simulink model "Highway_Assist"  (R2021a)
settings: Solver=VariableStepAuto  StartTime=0.0  StopTime=100  RelTol=1e-3
values from neighbouring files (symbols this model uses):
  Cf = 155494.663    [Highway_Assist_init.m]
  Cr = 1554494.663    [Highway_Assist_init.m]
  Iz = 1436.24    [Highway_Assist_init.m]
  lf = 1.165    [Highway_Assist_init.m]
  lr = 1.165    [Highway_Assist_init.m]
  m = 1140    [Highway_Assist_init.m]
  md = get_curvature(Vx, yaw_rate_pose, tRef)    [Highway_Assist_init.m]
  Ts = 0.1    [Highway_Assist_init.m]
  V_init = Vx    (= 25)    [Highway_Assist_init.m]
undefined symbols (not defined in the file or in its folder): sigbuilder_block
libraries: pid_lib x2, mpcadaslib x1
(part 1 of 2)
settings Model: Creator=User  LastModifiedBy=User

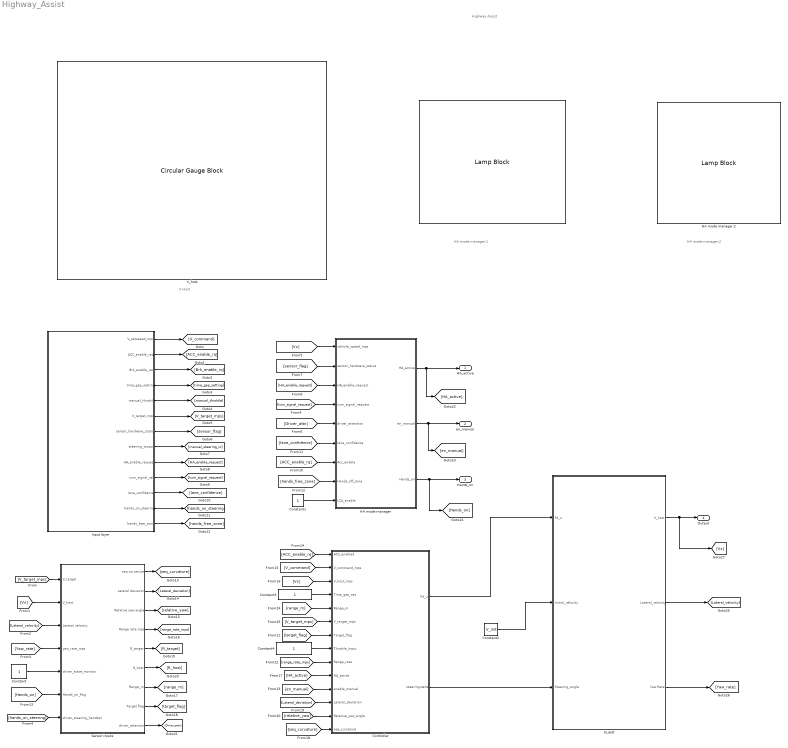
== system Highway_Assist ==
  note: HA mode manager:2
  note: V Host
  note: HA mode manager:1
  note: Highway Assist
  " " : LampBlock
  Constant{,1,3..4} (4 alike) : Constant
  Constant2 : Constant  Value=V_init
  Controller : Subsystem
  HA mode manager : Subsystem
  HA mode manager:2 : LampBlock
  Input layer : Subsystem
  PLANT : Subsystem
  Sensor inputs : Subsystem
  V_host : CircularGaugeBlock
  HA_active : Outport
  en_manual : Outport  Port=2
  Hands_on : Outport  Port=3
  Output : Outport  Port=4
  wires:
  Input layer/1(V_setspeed_mps) -> [V_command]
  Input layer/2(ACC_enable_req) -> [ACC_enable_rq]
  Input layer/3(Brk_enable_req) -> [Brk_enable_rq]
  Input layer/4(time_gap_setting) -> [time_gap_setting]
  Input layer/5(manual_throttle) -> [manual_throttle]
  Input layer/6(V_target_mps) -> [V_target_mps]
  Input layer/7(sensor_hardware_status) -> [sensor_flag]
  Input layer/8(steering_torque) -> [manual_steering_io]
  Input layer/9(HA_enable_request) -> [HA_enable_request]
  Input layer/10(turn_signal_req) -> [turn_signal_request]
  Input layer/11(lane_confidence) -> [lane_confidence]
  Input layer/12(hands_on_steering) -> [hands_on_steering]
  Input layer/13(hands_free_zone) -> [hands_free_zone]
  [V_target_mps] -> Sensor inputs/1(V_target)
  [Vx] -> Sensor inputs/2(V_host)
  [Lateral_velocity] -> Sensor inputs/3(Lateral velocity)
  [Yaw_rate] -> Sensor inputs/4(yaw_rate_mps)
  Constant/1 -> Sensor inputs/5(driver_state_monitor)
  [hands_on_steering] -> Sensor inputs/7(driver_steering_handson)
  [Vx] -> HA mode manager/1(vehicle_speed_mps)
  Sensor inputs/1(seq curvature) -> [seq_curvature]
  Sensor inputs/2(Lateral deviation) -> [Lateral_deviation]
  Sensor inputs/3(Relative yaw angle) -> [relative_yaw]
  Sensor inputs/4(Range rate mps) -> [range_rate_mps]
  Sensor inputs/7(Range_m) -> [range_m]
  Sensor inputs/8(Target flag) -> [target_flag]
  Sensor inputs/5(R_target) -> [R_target]
  Sensor inputs/6(R_host) -> [R_host]
  Sensor inputs/9(driver_attention) -> [Driver_attn]
  [Driver_attn] -> HA mode manager/5(driver_attention)
  [sensor_flag] -> HA mode manager/2(sensor_hardware_status)
  [HA_enable_request] -> HA mode manager/3(HA_enable_request)
  [turn_signal_request] -> HA mode manager/4(turn_signal_request)
  Constant1/1 -> HA mode manager/9(LCA_enable)
  [ACC_enable_rq] -> HA mode manager/7(Acc_enable)
  [lane_confidence] -> HA mode manager/6(lane_confidence)
  [hands_free_zone] -> HA mode manager/8(Hands_off_zone)
  HA mode manager/1(HA_active) -> [HA_active], HA_active/1
  HA mode manager/2(en_manual) -> [en_manual], en_manual/1
  HA mode manager/3(Hands_on) -> [Hands_on], Hands_on/1
  [Hands_on] -> Sensor inputs/6(Hands_on_flag)
  [ACC_enable_rq] -> Controller/1(ACC_enabled)
  [V_command] -> Controller/2(V_command_mps)
  [Vx] -> Controller/3(V_host_mps)
  Controller/1(Fd_u) -> PLANT/1(Fd_u)
  Controller/2(steering-delta) -> PLANT/3(Steering_angle)
  Constant2/1 -> PLANT/2(Initial_velocity)
  [HA_active] -> Controller/10(HA_active)
  [seq_curvature] -> Controller/14(seq_curvature)
  [Lateral_deviation] -> Controller/12(Lateral_deviation)
  [relative_yaw] -> Controller/13(Relative_yaw_angle)
  [target_flag] -> Controller/7(Target_flag)
  [range_rate_mps] -> Controller/9(Range_rate)
  [en_manual] -> Controller/11(enable_manual)
  [range_m] -> Controller/5(Range_m)
  [V_target_mps] -> Controller/6(V_target_mps)
  PLANT/2(Lateral_velocity) -> [Lateral_velocity]
  PLANT/3(Yaw Rate) -> [Yaw_rate]
  PLANT/1(V_host) -> Output/1, [Vx]
  Constant3/1 -> Controller/4(Time_gap_sec)
  Constant4/1 -> Controller/8(Throttle_input)

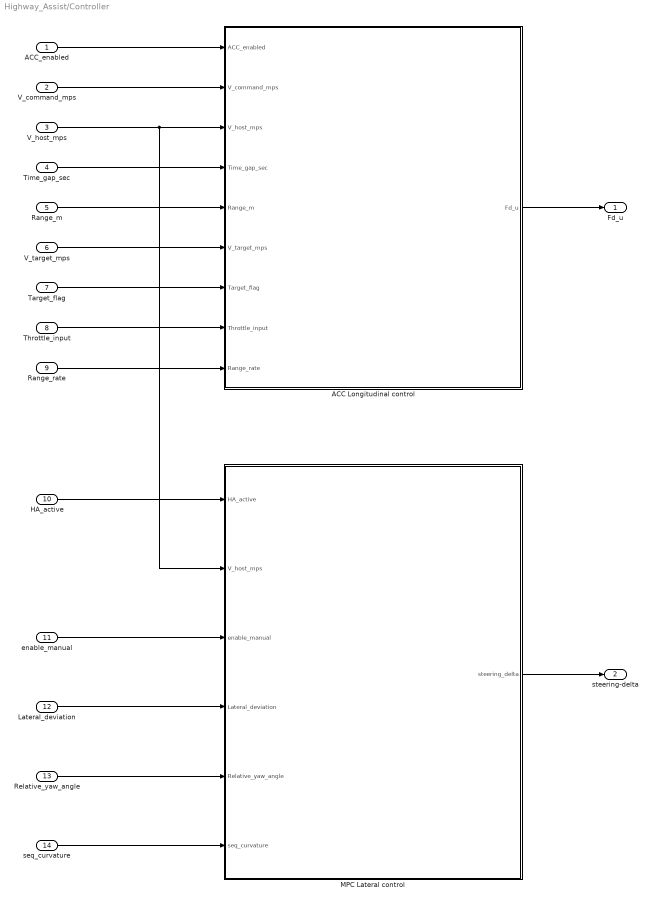
== system Highway_Assist/Controller ==
  ACC_enabled : Inport
  V_command_mps : Inport  Port=2
  V_host_mps : Inport  Port=3
  Time_gap_sec : Inport  Port=4
  Range_m : Inport  Port=5
  V_target_mps : Inport  Port=6
  Target_flag : Inport  Port=7
  Throttle_input : Inport  Port=8
  Range_rate : Inport  Port=9
  HA_active : Inport  Port=10
  enable_manual : Inport  Port=11
  Lateral_deviation : Inport  Port=12
  Relative_yaw_angle : Inport  Port=13
  seq_curvature : Inport  Port=14
  ACC Longitudinal control : Subsystem
  MPC Lateral control : Subsystem
  Fd_u : Outport
  steering-delta : Outport  Port=2
  wires:
  ACC_enabled/1 -> ACC Longitudinal control/1(ACC_enabled)
  V_command_mps/1 -> ACC Longitudinal control/2(V_command_mps)
  Time_gap_sec/1 -> ACC Longitudinal control/4(Time_gap_sec)
  Range_m/1 -> ACC Longitudinal control/5(Range_m)
  V_target_mps/1 -> ACC Longitudinal control/6(V_target_mps)
  Target_flag/1 -> ACC Longitudinal control/7(Target_flag)
  Throttle_input/1 -> ACC Longitudinal control/8(Throttle_input)
  Range_rate/1 -> ACC Longitudinal control/9(Range_rate)
  ACC Longitudinal control/1(Fd_u) -> Fd_u/1
  MPC Lateral control/1(steering_delta) -> steering-delta/1
  V_host_mps/1 -> MPC Lateral control/2(V_host_mps), ACC Longitudinal control/3(V_host_mps)
  HA_active/1 -> MPC Lateral control/1(HA_active)
  enable_manual/1 -> MPC Lateral control/3(enable_manual)
  Lateral_deviation/1 -> MPC Lateral control/4(Lateral_deviation)
  Relative_yaw_angle/1 -> MPC Lateral control/5(Relative_yaw_angle)
  seq_curvature/1 -> MPC Lateral control/6(seq_curvature)

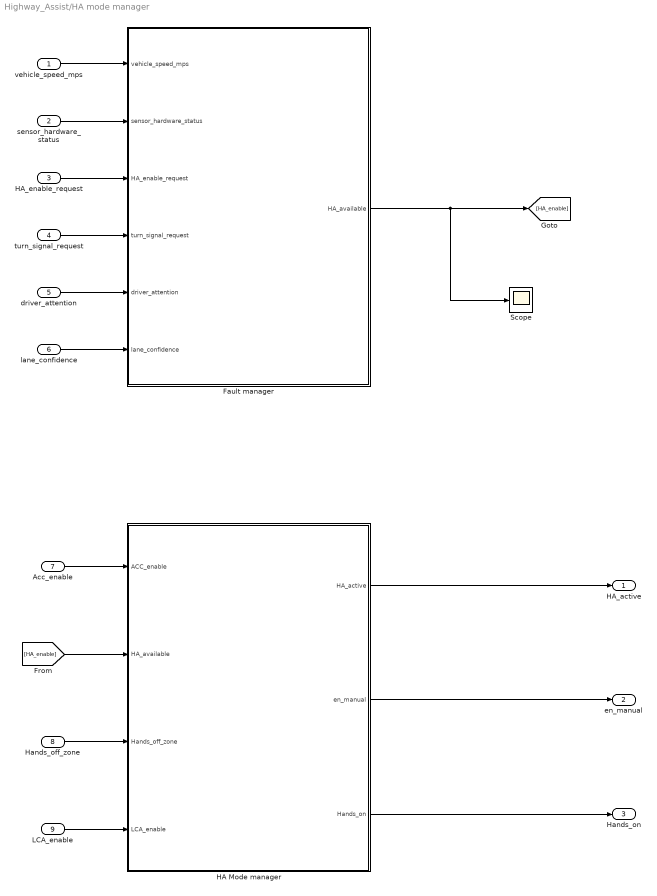
== system Highway_Assist/HA mode manager ==
  vehicle_speed_mps : Inport
  sensor_hardware_status : Inport  Port=2
  HA_enable_request : Inport  Port=3
  turn_signal_request : Inport  Port=4
  driver_attention : Inport  Port=5
  lane_confidence : Inport  Port=6
  Acc_enable : Inport  Port=7
  Hands_off_zone : Inport  Port=8
  LCA_enable : Inport  Port=9
  Fault manager : Subsystem
  HA Mode manager : Subsystem
  Scope : Scope
  HA_active : Outport
  en_manual : Outport  Port=2
  Hands_on : Outport  Port=3
  wires:
  vehicle_speed_mps/1 -> Fault manager/1(vehicle_speed_mps)
  sensor_hardware_status/1 -> Fault manager/2(sensor_hardware_status)
  HA_enable_request/1 -> Fault manager/3("\tHA_enable_request")
  turn_signal_request/1 -> Fault manager/4("\tturn_signal_request")
  driver_attention/1 -> Fault manager/5("\tdriver_attention")
  lane_confidence/1 -> Fault manager/6("\tlane_confidence")
  Acc_enable/1 -> HA Mode manager/1(ACC_enable)
  [HA_enable] -> HA Mode manager/2(HA_available)
  Hands_off_zone/1 -> HA Mode manager/3(Hands_off_zone)
  LCA_enable/1 -> HA Mode manager/4(LCA_enable)
  HA Mode manager/1(HA_active) -> HA_active/1
  HA Mode manager/2(en_manual) -> en_manual/1
  HA Mode manager/3(Hands_on) -> Hands_on/1
  Fault manager/1(HA_available) -> Scope/1, [HA_enable]

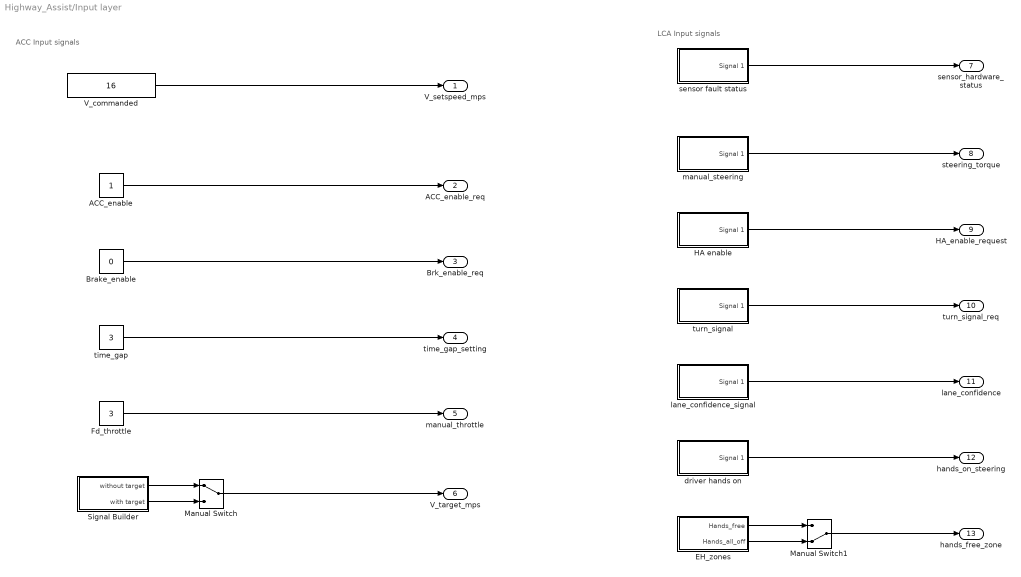
== system Highway_Assist/Input layer ==
  note: LCA Input signals
  note: ACC Input signals
  ACC_enable : Constant
  Brake_enable : Constant  Value=0
  EH_zones : Subsystem  Tag=STV Subsys  LoadFcn=sigbuilder_block('load');  StartFcn=sigbuilder_block('start');  StopFcn=sigbuilder_block('stop');  ClipboardFcn=sigbuilder_block('clipboard');  mask(Sigbuilder block){tuvar=[0:10]}
      mask help: Simulink:masks:SigbuilderBlock_MD
      mask init:
      | if ~strcmp(get_param(bdroot(gcbh),'SimulationStatus'),'stopped') tuvar = sigbuilder_block('maskInit'); end
      settings: CopyFcn=sigbuilder_block('copy');  DeleteFcn=sigbuilder_block('delete');  ModelCloseFcn=sigbuilder_block('modelClose');  PreSaveFcn=sigbuilder_block('preSave');  PauseFcn=sigbuilder_block('pause');  ContinueFcn=sigbuilder_block('continue');  NameChangeFcn=sigbuilder_block('namechange');  OpenFcn=sigbuilder_block('open',[320.25 248.25 550.5 359.25 ]);  CloseFcn=sigbuilder_block('close');
      mask Display: plot(0, 0, 100, 100,[2, 2, 32, 32, 2], [68, 8, 8, 68, 68],[32, 2], [38, 38], [32, 19, 2],[53, 60, 44], [32, 17, 17, 2],[16, 16, 31, 31]);txt = getActiveGroup(gcbh);text(2, 100, txt,'verticalAlignment', 'top');
  Fd_throttle : Constant  Value=3
  HA enable : Subsystem  Tag=STV Subsys  LoadFcn=sigbuilder_block('load');  StartFcn=sigbuilder_block('start');  StopFcn=sigbuilder_block('stop');  ClipboardFcn=sigbuilder_block('clipboard');  mask(Sigbuilder block){tuvar=[0:10]}
      mask help: Simulink:masks:SigbuilderBlock_MD
      mask init:
      | if ~strcmp(get_param(bdroot(gcbh),'SimulationStatus'),'stopped') tuvar = sigbuilder_block('maskInit'); end
      settings: CopyFcn=sigbuilder_block('copy');  DeleteFcn=sigbuilder_block('delete');  ModelCloseFcn=sigbuilder_block('modelClose');  PreSaveFcn=sigbuilder_block('preSave');  PauseFcn=sigbuilder_block('pause');  ContinueFcn=sigbuilder_block('continue');  NameChangeFcn=sigbuilder_block('namechange');  OpenFcn=sigbuilder_block('open',[437.6 199.2 550.4 400 ]);  CloseFcn=sigbuilder_block('close');
      mask Display: plot(0, 0, 100, 100,[2, 2, 32, 32, 2], [68, 8, 8, 68, 68],[32, 2], [38, 38], [32, 19, 2],[53, 60, 44], [32, 17, 17, 2],[16, 16, 31, 31]);txt = getActiveGroup(gcbh);text(2, 100, txt,'verticalAlignment', 'top');
  Manual Switch : ManualSwitch
  Manual Switch1 : ManualSwitch  CurrentSetting=0
  Signal Builder : Subsystem  Tag=STV Subsys  LoadFcn=sigbuilder_block('load');  StartFcn=sigbuilder_block('start');  StopFcn=sigbuilder_block('stop');  ClipboardFcn=sigbuilder_block('clipboard');  mask(Sigbuilder block){tuvar=[0:10]}
      mask help: Simulink:masks:SigbuilderBlock_MD
      mask init:
      | if ~strcmp(get_param(bdroot(gcbh),'SimulationStatus'),'stopped') tuvar = sigbuilder_block('maskInit'); end
      settings: CopyFcn=sigbuilder_block('copy');  DeleteFcn=sigbuilder_block('delete');  ModelCloseFcn=sigbuilder_block('modelClose');  PreSaveFcn=sigbuilder_block('preSave');  PauseFcn=sigbuilder_block('pause');  ContinueFcn=sigbuilder_block('continue');  NameChangeFcn=sigbuilder_block('namechange');  OpenFcn=sigbuilder_block('open',[299.25 217.5 550.5 359.25 ]);  CloseFcn=sigbuilder_block('close');
      mask Display: plot(0, 0, 100, 100,[2, 2, 32, 32, 2], [68, 8, 8, 68, 68],[32, 2], [38, 38], [32, 19, 2],[53, 60, 44], [32, 17, 17, 2],[16, 16, 31, 31]);txt = getActiveGroup(gcbh);text(2, 100, txt,'verticalAlignment', 'top');
  V_commanded : Constant  Value=16
  driver hands on : Subsystem  Tag=STV Subsys  LoadFcn=sigbuilder_block('load');  StartFcn=sigbuilder_block('start');  StopFcn=sigbuilder_block('stop');  ClipboardFcn=sigbuilder_block('clipboard');  mask(Sigbuilder block){tuvar=[0:10]}
      mask help: Simulink:masks:SigbuilderBlock_MD
      mask init:
      | if ~strcmp(get_param(bdroot(gcbh),'SimulationStatus'),'stopped') tuvar = sigbuilder_block('maskInit'); end
      settings: CopyFcn=sigbuilder_block('copy');  DeleteFcn=sigbuilder_block('delete');  ModelCloseFcn=sigbuilder_block('modelClose');  PreSaveFcn=sigbuilder_block('preSave');  PauseFcn=sigbuilder_block('pause');  ContinueFcn=sigbuilder_block('continue');  NameChangeFcn=sigbuilder_block('namechange');  OpenFcn=sigbuilder_block('open',[403.5 199.2 550.5 359.55 ]);  CloseFcn=sigbuilder_block('close');
      mask Display: plot(0, 0, 100, 100,[2, 2, 32, 32, 2], [68, 8, 8, 68, 68],[32, 2], [38, 38], [32, 19, 2],[53, 60, 44], [32, 17, 17, 2],[16, 16, 31, 31]);txt = getActiveGroup(gcbh);text(2, 100, txt,'verticalAlignment', 'top');
  lane_confidence_signal : Subsystem  Tag=STV Subsys  LoadFcn=sigbuilder_block('load');  StartFcn=sigbuilder_block('start');  StopFcn=sigbuilder_block('stop');  ClipboardFcn=sigbuilder_block('clipboard');  mask(Sigbuilder block){tuvar=[0:10]}
      mask help: Simulink:masks:SigbuilderBlock_MD
      mask init:
      | if ~strcmp(get_param(bdroot(gcbh),'SimulationStatus'),'stopped') tuvar = sigbuilder_block('maskInit'); end
      settings: CopyFcn=sigbuilder_block('copy');  DeleteFcn=sigbuilder_block('delete');  ModelCloseFcn=sigbuilder_block('modelClose');  PreSaveFcn=sigbuilder_block('preSave');  PauseFcn=sigbuilder_block('pause');  ContinueFcn=sigbuilder_block('continue');  NameChangeFcn=sigbuilder_block('namechange');  OpenFcn=sigbuilder_block('open',[437.6 199.2 550.4 400 ]);  CloseFcn=sigbuilder_block('close');
      mask Display: plot(0, 0, 100, 100,[2, 2, 32, 32, 2], [68, 8, 8, 68, 68],[32, 2], [38, 38], [32, 19, 2],[53, 60, 44], [32, 17, 17, 2],[16, 16, 31, 31]);txt = getActiveGroup(gcbh);text(2, 100, txt,'verticalAlignment', 'top');
  manual_steering : Subsystem  Tag=STV Subsys  LoadFcn=sigbuilder_block('load');  StartFcn=sigbuilder_block('start');  StopFcn=sigbuilder_block('stop');  ClipboardFcn=sigbuilder_block('clipboard');  mask(Sigbuilder block){tuvar=[0:10]}
      mask help: Simulink:masks:SigbuilderBlock_MD
      mask init:
      | if ~strcmp(get_param(bdroot(gcbh),'SimulationStatus'),'stopped') tuvar = sigbuilder_block('maskInit'); end
      settings: CopyFcn=sigbuilder_block('copy');  DeleteFcn=sigbuilder_block('delete');  ModelCloseFcn=sigbuilder_block('modelClose');  PreSaveFcn=sigbuilder_block('preSave');  PauseFcn=sigbuilder_block('pause');  ContinueFcn=sigbuilder_block('continue');  NameChangeFcn=sigbuilder_block('namechange');  OpenFcn=sigbuilder_block('open',[437.6 199.2 550.4 400 ]);  CloseFcn=sigbuilder_block('close');
      mask Display: plot(0, 0, 100, 100,[2, 2, 32, 32, 2], [68, 8, 8, 68, 68],[32, 2], [38, 38], [32, 19, 2],[53, 60, 44], [32, 17, 17, 2],[16, 16, 31, 31]);txt = getActiveGroup(gcbh);text(2, 100, txt,'verticalAlignment', 'top');
  sensor fault status : Subsystem  Tag=STV Subsys  LoadFcn=sigbuilder_block('load');  StartFcn=sigbuilder_block('start');  StopFcn=sigbuilder_block('stop');  ClipboardFcn=sigbuilder_block('clipboard');  mask(Sigbuilder block){tuvar=[0:10]}
      mask help: Simulink:masks:SigbuilderBlock_MD
      mask init:
      | if ~strcmp(get_param(bdroot(gcbh),'SimulationStatus'),'stopped') tuvar = sigbuilder_block('maskInit'); end
      settings: CopyFcn=sigbuilder_block('copy');  DeleteFcn=sigbuilder_block('delete');  ModelCloseFcn=sigbuilder_block('modelClose');  PreSaveFcn=sigbuilder_block('preSave');  PauseFcn=sigbuilder_block('pause');  ContinueFcn=sigbuilder_block('continue');  NameChangeFcn=sigbuilder_block('namechange');  OpenFcn=sigbuilder_block('open',[403.5 199.2 550.5 359.55 ]);  CloseFcn=sigbuilder_block('close');
      mask Display: plot(0, 0, 100, 100,[2, 2, 32, 32, 2], [68, 8, 8, 68, 68],[32, 2], [38, 38], [32, 19, 2],[53, 60, 44], [32, 17, 17, 2],[16, 16, 31, 31]);txt = getActiveGroup(gcbh);text(2, 100, txt,'verticalAlignment', 'top');
  time_gap : Constant  Value=3
  turn_signal : Subsystem  Tag=STV Subsys  LoadFcn=sigbuilder_block('load');  StartFcn=sigbuilder_block('start');  StopFcn=sigbuilder_block('stop');  ClipboardFcn=sigbuilder_block('clipboard');  mask(Sigbuilder block){tuvar=[0:10]}
      mask help: Simulink:masks:SigbuilderBlock_MD
      mask init:
      | if ~strcmp(get_param(bdroot(gcbh),'SimulationStatus'),'stopped') tuvar = sigbuilder_block('maskInit'); end
      settings: CopyFcn=sigbuilder_block('copy');  DeleteFcn=sigbuilder_block('delete');  ModelCloseFcn=sigbuilder_block('modelClose');  PreSaveFcn=sigbuilder_block('preSave');  PauseFcn=sigbuilder_block('pause');  ContinueFcn=sigbuilder_block('continue');  NameChangeFcn=sigbuilder_block('namechange');  OpenFcn=sigbuilder_block('open',[437.6 199.2 550.4 400 ]);  CloseFcn=sigbuilder_block('close');
      mask Display: plot(0, 0, 100, 100,[2, 2, 32, 32, 2], [68, 8, 8, 68, 68],[32, 2], [38, 38], [32, 19, 2],[53, 60, 44], [32, 17, 17, 2],[16, 16, 31, 31]);txt = getActiveGroup(gcbh);text(2, 100, txt,'verticalAlignment', 'top');
  V_setspeed_mps : Outport
  ACC_enable_req : Outport  Port=2
  Brk_enable_req : Outport  Port=3
  time_gap_setting : Outport  Port=4
  manual_throttle : Outport  Port=5
  V_target_mps : Outport  Port=6
  sensor_hardware_status : Outport  Port=7
  steering_torque : Outport  Port=8
  HA_enable_request : Outport  Port=9
  turn_signal_req : Outport  Port=10
  lane_confidence : Outport  Port=11
  hands_on_steering : Outport  Port=12
  hands_free_zone : Outport  Port=13
  wires:
  V_commanded/1 -> V_setspeed_mps/1
  ACC_enable/1 -> ACC_enable_req/1
  Brake_enable/1 -> Brk_enable_req/1
  time_gap/1 -> time_gap_setting/1
  Fd_throttle/1 -> manual_throttle/1
  Signal Builder/1(without target) -> Manual Switch/1
  Signal Builder/2(with target) -> Manual Switch/2
  Manual Switch/1 -> V_target_mps/1
  sensor fault status/1(Signal 1) -> sensor_hardware_status/1
  manual_steering/1(Signal 1) -> steering_torque/1
  HA enable/1(Signal 1) -> HA_enable_request/1
  turn_signal/1(Signal 1) -> turn_signal_req/1
  lane_confidence_signal/1(Signal 1) -> lane_confidence/1
  driver hands on/1(Signal 1) -> hands_on_steering/1
  Manual Switch1/1 -> hands_free_zone/1
  EH_zones/2(Hands_all_off) -> Manual Switch1/2
  EH_zones/1(Hands_free) -> Manual Switch1/1

== system Highway_Assist/PLANT ==
  Fd_u : Inport
  Initial_velocity : Inport  Port=2
  Steering_angle : Inport  Port=3
  Lateral Vehicle Dynamics : Subsystem
  Longitudinal Vehicle Dynamics : Subsystem
  Scope : Scope
  V_host : Outport
  Lateral_velocity : Outport  Port=2  Unit=m/s  VectorParamsAs1DForOutWhenUnconnected=off
  Yaw Rate : Outport  Port=3  Unit=degree/s  VectorParamsAs1DForOutWhenUnconnected=off
  wires:
  Longitudinal Vehicle Dynamics/1(V_host) -> Scope/1, V_host/1, Lateral Vehicle Dynamics/1(Longitudinal velocity)
  Steering_angle/1 -> Lateral Vehicle Dynamics/2(Steering angle)
  Lateral Vehicle Dynamics/1(Lateral Velocity) -> Lateral_velocity/1
  Lateral Vehicle Dynamics/2(Yaw Rate) -> Yaw Rate/1
  Fd_u/1 -> Longitudinal Vehicle Dynamics/1(Fd_u)
  Initial_velocity/1 -> Longitudinal Vehicle Dynamics/2(initial_velocity)

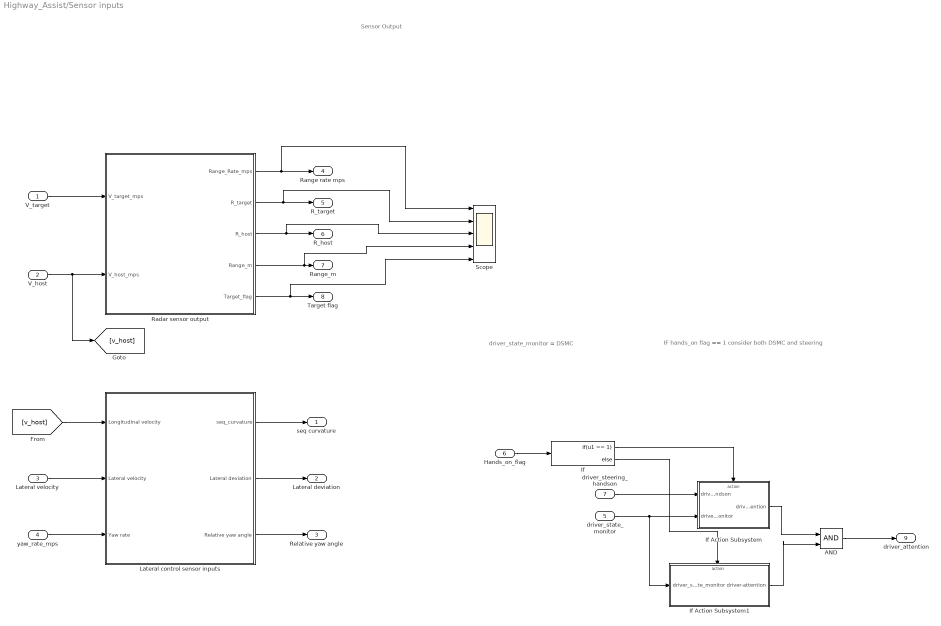
== system Highway_Assist/Sensor inputs ==
  note: IF hands_on flag == 1 consider both DSMC and steering
  note: driver_state_monitor = DSMC
  note: Sensor Output
  V_target : Inport
  V_host : Inport  Port=2
  Lateral velocity : Inport  Port=3
  yaw_rate_mps : Inport  Port=4
  driver_state_monitor : Inport  Port=5
  Hands_on_flag : Inport  Port=6
  driver_steering_handson : Inport  Port=7
  AND : Logic  IconShape=distinctive  AllPortsSameDT=off  OutDataTypeStr=boolean
  If : If  IfExpression=u1 == 1
  If Action Subsystem : Subsystem  TreatAsAtomicUnit=on
  If Action Subsystem1 : Subsystem  TreatAsAtomicUnit=on
  Lateral control sensor inputs : Subsystem
  Radar sensor output : Subsystem
  Scope : Scope  NumInputPorts=5
  seq curvature : Outport
  Lateral deviation : Outport  Port=2
  Relative yaw angle : Outport  Port=3
  Range rate mps : Outport  Port=4
  R_target : Outport  Port=5
  R_host : Outport  Port=6
  Range_m : Outport  Port=7
  Target flag : Outport  Port=8
  driver_attention : Outport  Port=9
  wires:
  V_target/1 -> Radar sensor output/1(V_target_mps)
  V_host/1 -> [v_host], Radar sensor output/2(V_host_mps)
  [v_host] -> Lateral control sensor inputs/1(Longitudinal velocity)
  Lateral velocity/1 -> Lateral control sensor inputs/2(Lateral velocity)
  yaw_rate_mps/1 -> Lateral control sensor inputs/3(Yaw rate)
  Lateral control sensor inputs/3(Relative yaw angle) -> Relative yaw angle/1
  Lateral control sensor inputs/2(Lateral deviation) -> Lateral deviation/1
  Lateral control sensor inputs/1(seq_curvature) -> seq curvature/1
  Radar sensor output/5(Target_flag) -> Scope/5, Target flag/1
  Radar sensor output/4(Range_m) -> Scope/4, Range_m/1
  Radar sensor output/3(R_host) -> Scope/3, R_host/1
  Radar sensor output/2(R_target) -> Scope/2, R_target/1
  Radar sensor output/1(Range_Rate_mps) -> Scope/1, Range rate mps/1
  Hands_on_flag/1 -> If/1
  If/1 -> If Action Subsystem/Action
  If/2 -> If Action Subsystem1/Action
  If Action Subsystem/1(driver-attention) -> AND/1
  If Action Subsystem1/1(driver-attention) -> AND/2
  AND/1 -> driver_attention/1
  driver_steering_handson/1 -> If Action Subsystem/1(driver_steering_handson)
  driver_state_monitor/1 -> If Action Subsystem1/1(driver_state_monitor), If Action Subsystem/2(driver_state_monitor)

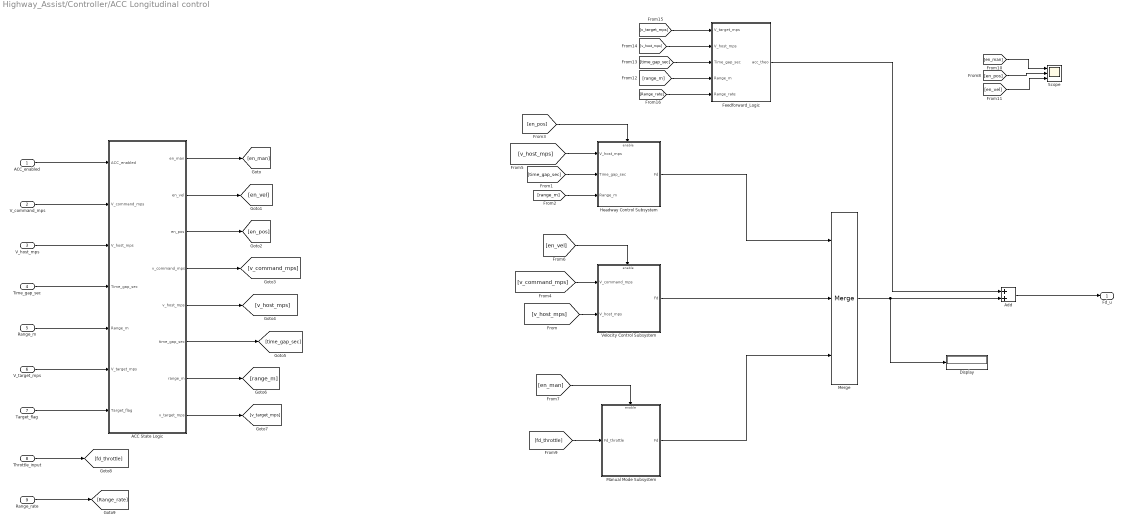
== system Highway_Assist/Controller/ACC Longitudinal control ==
  ACC_enabled : Inport
  V_command_mps : Inport  Port=2
  V_host_mps : Inport  Port=3
  Time_gap_sec : Inport  Port=4
  Range_m : Inport  Port=5
  V_target_mps : Inport  Port=6
  Target_flag : Inport  Port=7
  Throttle_input : Inport  Port=8
  Range_rate : Inport  Port=9
  ACC State Logic : Subsystem
  Add : Sum
  Display : Display
  Feedforward_Logic : Subsystem
  Headway Control Subsystem : Subsystem
  Manual Mode Subsystem : Subsystem
  Merge : Merge  Inputs=3
  Scope : Scope  NumInputPorts=3
  Velocity Control Subsystem : Subsystem
  Fd_u : Outport
  wires:
  ACC State Logic/3(en_pos) -> [en_pos]
  ACC_enabled/1 -> ACC State Logic/1(ACC_enabled)
  ACC State Logic/2(en_vel) -> [en_vel]
  Target_flag/1 -> ACC State Logic/7(Target_flag)
  ACC State Logic/8(v_target_mps) -> [v_target_mps]
  V_target_mps/1 -> ACC State Logic/6(V_target_mps)
  Time_gap_sec/1 -> ACC State Logic/4(Time_gap_sec)
  Range_m/1 -> ACC State Logic/5(Range_m)
  ACC State Logic/6(time_gap_sec) -> [time_gap_sec]
  ACC State Logic/4(v_command_mps) -> [v_command_mps]
  V_command_mps/1 -> ACC State Logic/2(V_command_mps)
  V_host_mps/1 -> ACC State Logic/3(V_host_mps)
  ACC State Logic/5(v_host_mps) -> [v_host_mps]
  ACC State Logic/7(range_m) -> [range_m]
  ACC State Logic/1(en_man) -> [en_man]
  [v_host_mps] -> Velocity Control Subsystem/2(V_host_mps)
  [en_vel] -> Scope/3
  [en_man] -> Scope/1
  [fd_throttle] -> Manual Mode Subsystem/1(Fd_throttle)
  Manual Mode Subsystem/1(Fd) -> Merge/3
  Headway Control Subsystem/1(Fd) -> Merge/1
  Velocity Control Subsystem/1(Fd) -> Merge/2
  Feedforward_Logic/1(acc_theo) -> Add/1
  [en_vel] -> Velocity Control Subsystem/Enable
  [range_m] -> Headway Control Subsystem/3(Range_m)
  [en_man] -> Manual Mode Subsystem/Enable
  [range_m] -> Feedforward_Logic/4(Range_m)
  [time_gap_sec] -> Feedforward_Logic/3(Time_gap_sec)
  [v_host_mps] -> Feedforward_Logic/2(V_host_mps)
  [time_gap_sec] -> Headway Control Subsystem/2(Time_gap_sec)
  [v_target_mps] -> Feedforward_Logic/1(V_target_mps)
  [v_host_mps] -> Headway Control Subsystem/1(V_host_mps)
  Merge/1 -> Add/2, Display/1
  [en_pos] -> Scope/2
  [en_pos] -> Headway Control Subsystem/Enable
  Add/1 -> Fd_u/1
  [Range_rate] -> Feedforward_Logic/5(Range_rate)
  [v_command_mps] -> Velocity Control Subsystem/1(V_command_mps)
  Throttle_input/1 -> [fd_throttle]
  Range_rate/1 -> [Range_rate]

== system Highway_Assist/Controller/MPC Lateral control ==
  HA_active : Inport
  V_host_mps : Inport  Port=2
  enable_manual : Inport  Port=3
  Lateral_deviation : Inport  Port=4
  Relative_yaw_angle : Inport  Port=5
  seq_curvature : Inport  Port=6
  MPC : Subsystem
  Merge : Merge
  manual : Subsystem
  steering_delta : Outport
  wires:
  enable_manual/1 -> manual/Enable
  Lateral_deviation/1 -> MPC/3(lateral_deviation)
  Relative_yaw_angle/1 -> MPC/4(Relative_yaw_angle)
  Merge/1 -> steering_delta/1
  MPC/1(steering angle (rad)) -> Merge/1
  HA_active/1 -> MPC/Enable
  manual/1(delta) -> Merge/2
  V_host_mps/1 -> MPC/2(V_host_mps)
  seq_curvature/1 -> MPC/1(seq_curvature)

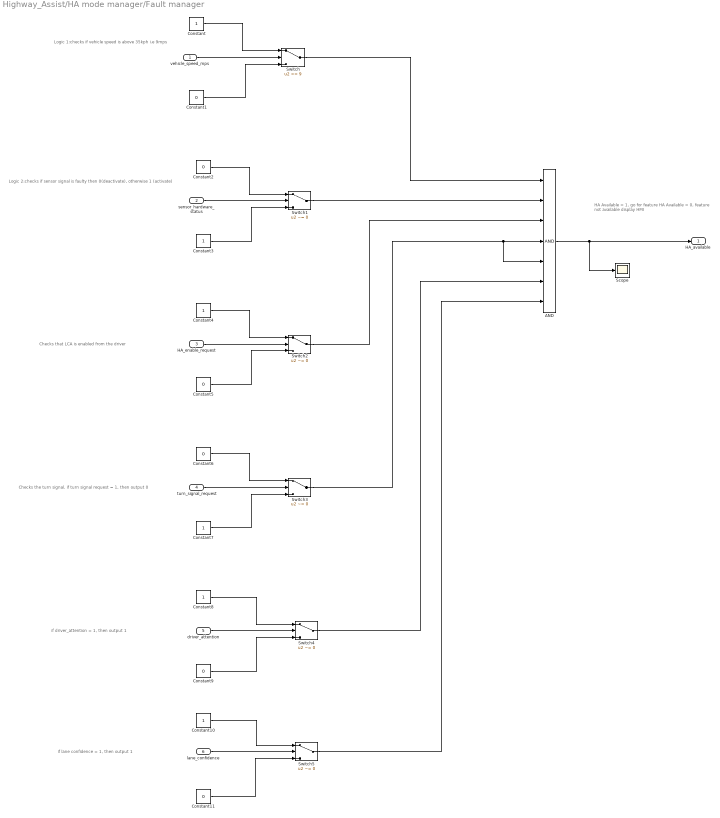
== system Highway_Assist/HA mode manager/Fault manager ==
  note: Logic 1:checks if vehicle speed is above 35kph i.e 9mps
  note: Logic 2:checks if sensor signal is faulty then 0(deactivate), otherwise 1 (activate)
  note: Checks that LCA is enabled from the driver
  note: Checks the turn signal. if turn signal request = 1, then output 0
  note: if driver_attention = 1, then output 1
  note: HA Available = 1, go for feature
      | HA Available = 0, feature not available display HMI
  note: if lane confidence = 1, then output 1
  vehicle_speed_mps : Inport
  sensor_hardware_status : Inport  Port=2
  "\tHA_enable_request" : Inport  Port=3
  "\tturn_signal_request" : Inport  Port=4
  "\tdriver_attention" : Inport  Port=5
  "\tlane_confidence" : Inport  Port=6
  AND : Logic  Inputs=7  AllPortsSameDT=off  OutDataTypeStr=boolean
  Constant{,3..4,7..8,10} (6 alike) : Constant
  Constant{1..2,5..6,9,11} (6 alike) : Constant  Value=0
  Scope : Scope
  Switch : Switch  Threshold=9
  Switch{1..5} (5 alike) : Switch  Criteria=u2 ~= 0
  HA_available : Outport
  wires:
  vehicle_speed_mps/1 -> Switch/2
  Constant/1 -> Switch/1
  Constant1/1 -> Switch/3
  Constant3/1 -> Switch1/3
  Constant2/1 -> Switch1/1
  sensor_hardware_status/1 -> Switch1/2
  "\tHA_enable_request"/1 -> Switch2/2
  Constant4/1 -> Switch2/1
  Constant5/1 -> Switch2/3
  Constant7/1 -> Switch3/3
  Constant6/1 -> Switch3/1
  "\tturn_signal_request"/1 -> Switch3/2
  "\tdriver_attention"/1 -> Switch4/2
  Constant8/1 -> Switch4/1
  Constant9/1 -> Switch4/3
  Switch/1 -> AND/1
  Switch1/1 -> AND/2
  Switch2/1 -> AND/3
  Switch3/1 -> AND/5, AND/4
  Switch4/1 -> AND/6
  AND/1 -> HA_available/1, Scope/1
  "\tlane_confidence"/1 -> Switch5/2
  Constant10/1 -> Switch5/1
  Constant11/1 -> Switch5/3
  Switch5/1 -> AND/7

== system Highway_Assist/HA mode manager/HA Mode manager ==
  ACC_enable : Inport
  HA_available : Inport  Port=2
  Hands_off_zone : Inport  Port=3
  LCA_enable : Inport  Port=4
  Chart : Stateflow chart  TreatAsAtomicUnit=on
  HA_active : Outport
  en_manual : Outport  Port=2
  Hands_on : Outport  Port=3
  wires:
  ACC_enable/1 -> Chart/1(ACC_enable)
  HA_available/1 -> Chart/2(HA_available)
  Hands_off_zone/1 -> Chart/3(Hands_off_zone)
  LCA_enable/1 -> Chart/4(LCA_enable)
  Chart/2(en_manual) -> en_manual/1
  Chart/1(HA_active) -> HA_active/1
  Chart/3(Hands_on) -> Hands_on/1

== system Highway_Assist/Input layer/EH_zones ==
  Demux : Demux  Tag=STV Demux  Outputs=2
      settings: DisplayOption=none
  FromWs : FromWorkspace  Tag=STV FromWs  VariableName=tuvar
      SigBuilderData=|
      | common.afterFinalStr = 'Extrapolate'
      | common.sampleTime = 0
      | dataSet.timeRange = [0 100]
      | dataSet.name = 'Group 1'
      | sbobj.Groups.Name = 'Group 1'
      | sbobj.Groups.Signals(1).Name = 'Hands_free'
      | sbobj.Groups.Signals(1).XData = [0 4 6 100]
      | sbobj.Groups.Signals(1).YData = [1 1 1 1]
      | sbobj.Groups.Signals(2).Name = 'Hands_all_off'
      | sbobj.Groups.Signals(2).XData = [0 50 50 100]
      | sbobj.Groups.Signals(2).YData = [0 0 1 1]
      | sbobj.Groups.TimeRange = [0 100]
  Hands_free : Outport  Tag=STV Outport
  Hands_all_off : Outport  Tag=STV Outport  Port=2
  wires:
  Demux/1 -> Hands_free/1
  FromWs/1 -> Demux/1
  Demux/2 -> Hands_all_off/1

== system Highway_Assist/Input layer/HA enable ==
  Demux : Demux  Tag=STV Demux  Outputs=1
      settings: DisplayOption=none
  FromWs : FromWorkspace  Tag=STV FromWs  VariableName=tuvar
      SigBuilderData=|
      | common.afterFinalStr = 'Extrapolate'
      | common.sampleTime = 0
      | dataSet.timeRange = [0 10]
      | dataSet.name = 'Group 1'
      | sbobj.Groups.Name = 'Group 1'
      | sbobj.Groups.Signals.Name = 'Signal 1'
      | sbobj.Groups.Signals.XData = [0 4 4 6 6 10]
      | sbobj.Groups.Signals.YData = [0 0 1 1 0 0]
  Signal 1 : Outport  Tag=STV Outport
  wires:
  Demux/1 -> Signal 1/1
  FromWs/1 -> Demux/1

== system Highway_Assist/Input layer/Signal Builder ==
  Demux : Demux  Tag=STV Demux  Outputs=2
      settings: DisplayOption=none
  FromWs : FromWorkspace  Tag=STV FromWs  VariableName=tuvar
      SigBuilderData=|
      | common.afterFinalStr = 'Extrapolate'
      | common.sampleTime = 0
      | dataSet.timeRange = [0 100]
      | dataSet.name = 'Group 1'
      | sbobj.Groups.Name = 'Group 1'
      | sbobj.Groups.Signals(1).Name = 'without target'
      | sbobj.Groups.Signals(1).XData = [0 100]
      | sbobj.Groups.Signals(1).YData = [0 0]
      | sbobj.Groups.Signals(2).Name = 'with target'
      | sbobj.Groups.Signals(2).XData = [0 8.5 8.5 100]
      | sbobj.Groups.Signals(2).YData = [27.5 27 10 10]
      | sbobj.Groups.TimeRange = [0 100]
  without target : Outport  Tag=STV Outport
  with target : Outport  Tag=STV Outport  Port=2
  wires:
  FromWs/1 -> Demux/1
  Demux/1 -> without target/1
  Demux/2 -> with target/1

== system Highway_Assist/Input layer/driver hands on ==
  Demux : Demux  Tag=STV Demux  Outputs=1
      settings: DisplayOption=none
  FromWs : FromWorkspace  Tag=STV FromWs  VariableName=tuvar
      SigBuilderData=|
      | common.afterFinalStr = 'Extrapolate'
      | common.sampleTime = 0
      | dataSet.timeRange = [0 10]
      | dataSet.name = 'Group 1'
      | sbobj.Groups.Name = 'Group 1'
      | sbobj.Groups.Signals.Name = 'Signal 1'
      | sbobj.Groups.Signals.XData = [0 4 6 6 10]
      | sbobj.Groups.Signals.YData = [1 1 1 1 1]
  Signal 1 : Outport  Tag=STV Outport
  wires:
  FromWs/1 -> Demux/1
  Demux/1 -> Signal 1/1

== system Highway_Assist/Input layer/lane_confidence_signal ==
  Demux : Demux  Tag=STV Demux  Outputs=1
      settings: DisplayOption=none
  FromWs : FromWorkspace  Tag=STV FromWs  VariableName=tuvar
      SigBuilderData=|
      | common.afterFinalStr = 'Extrapolate'
      | common.sampleTime = 0
      | dataSet.timeRange = [0 10]
      | dataSet.name = 'Group 1'
      | sbobj.Groups.Name = 'Group 1'
      | sbobj.Groups.Signals.Name = 'Signal 1'
      | sbobj.Groups.Signals.XData = [0 4 4 6 6 10]
      | sbobj.Groups.Signals.YData = [0 0 1 1 0 0]
  Signal 1 : Outport  Tag=STV Outport
  wires:
  Demux/1 -> Signal 1/1
  FromWs/1 -> Demux/1

== system Highway_Assist/Input layer/manual_steering ==
  Demux : Demux  Tag=STV Demux  Outputs=1
      settings: DisplayOption=none
  FromWs : FromWorkspace  Tag=STV FromWs  VariableName=tuvar
      SigBuilderData=|
      | common.afterFinalStr = 'Extrapolate'
      | common.sampleTime = 0
      | dataSet.timeRange = [0 10]
      | dataSet.name = 'Group 1'
      | sbobj.Groups.Name = 'Group 1'
      | sbobj.Groups.Signals.Name = 'Signal 1'
      | sbobj.Groups.Signals.XData = [0 4 4 6 6 10]
      | sbobj.Groups.Signals.YData = [0 0 1 1 0 0]
  Signal 1 : Outport  Tag=STV Outport
  wires:
  FromWs/1 -> Demux/1
  Demux/1 -> Signal 1/1

== system Highway_Assist/Input layer/sensor fault status ==
  Demux : Demux  Tag=STV Demux  Outputs=1
      settings: DisplayOption=none
  FromWs : FromWorkspace  Tag=STV FromWs  VariableName=tuvar
      SigBuilderData=|
      | common.afterFinalStr = 'Extrapolate'
      | common.sampleTime = 0
      | dataSet.timeRange = [0 10]
      | dataSet.name = 'Group 1'
      | sbobj.Groups.Name = 'Group 1'
      | sbobj.Groups.Signals.Name = 'Signal 1'
      | sbobj.Groups.Signals.XData = [0 4 6 10]
      | sbobj.Groups.Signals.YData = [0 0 0 0]
  Signal 1 : Outport  Tag=STV Outport
  wires:
  Demux/1 -> Signal 1/1
  FromWs/1 -> Demux/1

== system Highway_Assist/Input layer/turn_signal ==
  Demux : Demux  Tag=STV Demux  Outputs=1
      settings: DisplayOption=none
  FromWs : FromWorkspace  Tag=STV FromWs  VariableName=tuvar
      SigBuilderData=|
      | common.afterFinalStr = 'Extrapolate'
      | common.sampleTime = 0
      | dataSet.timeRange = [0 10]
      | dataSet.name = 'Group 1'
      | sbobj.Groups.Name = 'Group 1'
      | sbobj.Groups.Signals.Name = 'Signal 1'
      | sbobj.Groups.Signals.XData = [0 4 4 6 6 10]
      | sbobj.Groups.Signals.YData = [0 0 1 1 0 0]
  Signal 1 : Outport  Tag=STV Outport
  wires:
  FromWs/1 -> Demux/1
  Demux/1 -> Signal 1/1

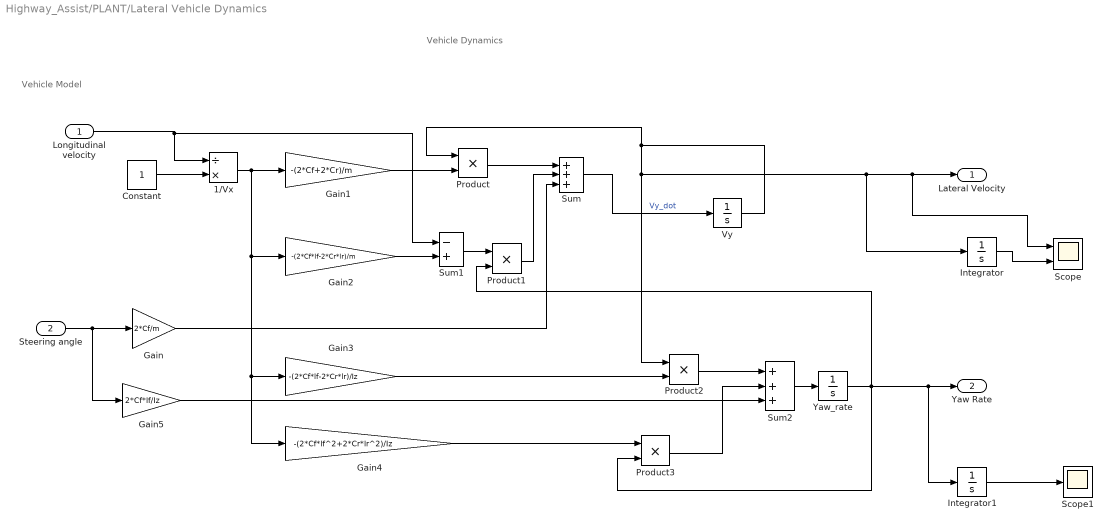
== system Highway_Assist/PLANT/Lateral Vehicle Dynamics ==
  note: Vehicle Model
  note: Vehicle Dynamics
  Longitudinal velocity : Inport
  Steering angle : Inport  Port=2
  1/Vx : Product  Inputs=/*
  Constant : Constant
  Gain : Gain  Gain=2*Cf/m
  Gain1 : Gain  Gain=-(2*Cf+2*Cr)/m
  Gain2 : Gain  Gain=-(2*Cf*lf-2*Cr*lr)/m
  Gain3 : Gain  Gain=-(2*Cf*lf-2*Cr*lr)/Iz
  Gain4 : Gain  Gain=-(2*Cf*lf^2+2*Cr*lr^2)/Iz
  Gain5 : Gain  Gain=2*Cf*lf/Iz
  Integrator : Integrator
  Integrator1 : Integrator
  Product{,1..3} (4 alike) : Product
  Scope : Scope  NumInputPorts=2
  Scope1 : Scope
  Sum : Sum  Inputs=+++
  Sum1 : Sum  Inputs=-+
  Sum2 : Sum  Inputs=+++
  Vy : Integrator
  "Yaw_rate " : Integrator
  Lateral Velocity : Outport  VectorParamsAs1DForOutWhenUnconnected=off
  Yaw Rate : Outport  Port=2  VectorParamsAs1DForOutWhenUnconnected=off
  wires:
  Sum2/1 -> "Yaw_rate "/1
  Gain2/1 -> Sum1/2
  Gain4/1 -> Product3/1
  Constant/1 -> 1/Vx/2
  Gain3/1 -> Product2/2
  1/Vx/1 -> Gain4/1, Gain3/1, Gain2/1, Gain1/1
  Product2/1 -> Sum2/1
  Product3/1 -> Sum2/2
  Gain5/1 -> Sum2/3
  Sum1/1 -> Product1/1
  "Yaw_rate "/1 -> Product3/2, Integrator1/1, Yaw Rate/1, Product1/2
  Gain/1 -> Sum/3
  Steering angle/1 -> Gain/1, Gain5/1
  Gain1/1 -> Product/2
  Product/1 -> Sum/1
  Vy/1 -> Product/1, Integrator/1, Scope/1, Lateral Velocity/1, Product2/1
  Sum/1 -> Vy/1  "Vy_dot"
  Longitudinal velocity/1 -> Sum1/1, 1/Vx/1
  Product1/1 -> Sum/2
  Integrator/1 -> Scope/2
  Integrator1/1 -> Scope1/1

== system Highway_Assist/PLANT/Longitudinal Vehicle Dynamics ==
  Fd_u : Inport
  initial_velocity : Inport  Port=2
  Add : Sum  Inputs=|+-
  Gain : Gain  Gain=9.211*1e-4
  Gain1 : Gain  Gain=0.2116
  Integrator : Integrator  InitialConditionSource=external
  V_host : Outport
  wires:
  Gain1/1 -> Add/2
  Fd_u/1 -> Gain/1
  Integrator/1 -> V_host/1, Gain1/1
  Add/1 -> Integrator/1
  initial_velocity/1 -> Integrator/2
  Gain/1 -> Add/1

== system Highway_Assist/Sensor inputs/If Action Subsystem ==
  driver_steering_handson : Inport
  driver_state_monitor : Inport  Port=2
  Action Port : ActionPort  ActionPortLabel=if(u1 == 1)
  AND : Logic  IconShape=distinctive  AllPortsSameDT=off  OutDataTypeStr=boolean
  driver-attention : Outport
  wires:
  driver_steering_handson/1 -> AND/1
  driver_state_monitor/1 -> AND/2
  AND/1 -> driver-attention/1

== system Highway_Assist/Sensor inputs/If Action Subsystem1 ==
  driver_state_monitor : Inport
  Action Port : ActionPort  ActionPortLabel=else
  driver-attention : Outport
  wires:
  driver_state_monitor/1 -> driver-attention/1

== system Highway_Assist/Sensor inputs/Lateral control sensor inputs ==
  note: Lateral Dynamics For MPC
  Longitudinal velocity : Inport
  Lateral velocity : Inport  Port=2
  Yaw rate : Inport  Port=3
  Subsystem : Subsystem  mask{signal=md, ts=Ts, steps=10}
      mask prompts: signal "Signal name"; ts "Sampling time"; steps "Number of previewing steps"
      mask init:
      | ts = evalin('base',get_param(gcbh,'ts'));
      | signal = evalin('base',get_param(gcbh,'signal'));
      | steps = evalin('base',get_param(gcbh,'steps'));
      | data = mpc_previewer_maskinit(signal,ts);
      mask Display:
      | fprintf('Future\nsample\nextractor');
      | port_label('output', 1, 'seq')
      | port_label('output', 2, '@t')
  sensor dynamics : Subsystem
  seq_curvature : Outport
  Lateral deviation : Outport  Port=2
  Relative yaw angle : Outport  Port=3
  wires:
  Yaw rate/1 -> sensor dynamics/4(Yaw rate)
  Lateral velocity/1 -> sensor dynamics/3(Lateral velocity)
  Longitudinal velocity/1 -> sensor dynamics/2(Longitudinal velocity)
  sensor dynamics/2(Relative yaw angle) -> Relative yaw angle/1
  sensor dynamics/1(Lateral deviation) -> Lateral deviation/1
  Subsystem/2(current) -> sensor dynamics/1(Current_curvature)
  Subsystem/1(sequence) -> seq_curvature/1

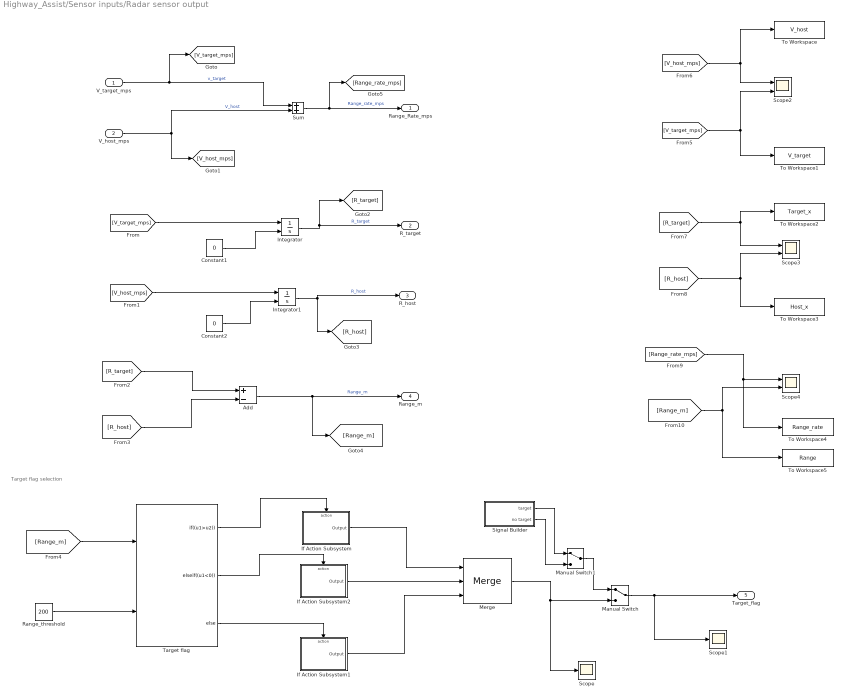
== system Highway_Assist/Sensor inputs/Radar sensor output ==
  note: Target flag selection
  V_target_mps : Inport
  V_host_mps : Inport  Port=2
  Add : Sum  Inputs=+-
  Constant1 : Constant  Value=0
  Constant2 : Constant  Value=0
  If Action Subsystem : Subsystem  TreatAsAtomicUnit=on
  If Action Subsystem1 : Subsystem  TreatAsAtomicUnit=on
  If Action Subsystem2 : Subsystem  TreatAsAtomicUnit=on
  Integrator : Integrator  InitialConditionSource=external  InitialCondition=500
  Integrator1 : Integrator  InitialConditionSource=external
  Manual Switch : ManualSwitch
  Manual Switch1 : ManualSwitch
  Merge : Merge  Inputs=3
  Range_threshold : Constant  Value=200
  Scope : Scope
  Scope1 : Scope
  Scope2 : Scope  NumInputPorts=2
  Scope3 : Scope  NumInputPorts=2
  Scope4 : Scope  NumInputPorts=2
  Signal Builder : Subsystem  Tag=STV Subsys  LoadFcn=sigbuilder_block('load');  StartFcn=sigbuilder_block('start');  StopFcn=sigbuilder_block('stop');  ClipboardFcn=sigbuilder_block('clipboard');  mask(Sigbuilder block){tuvar=[0:10]}
      mask help: Simulink:masks:SigbuilderBlock_MD
      mask init:
      | if ~strcmp(get_param(bdroot(gcbh),'SimulationStatus'),'stopped') tuvar = sigbuilder_block('maskInit'); end
      settings: CopyFcn=sigbuilder_block('copy');  DeleteFcn=sigbuilder_block('delete');  ModelCloseFcn=sigbuilder_block('modelClose');  PreSaveFcn=sigbuilder_block('preSave');  PauseFcn=sigbuilder_block('pause');  ContinueFcn=sigbuilder_block('continue');  NameChangeFcn=sigbuilder_block('namechange');  OpenFcn=sigbuilder_block('open',[234.75 201.75 550.5 359.25 ]);  CloseFcn=sigbuilder_block('close');
      mask Display: plot(0, 0, 100, 100,[2, 2, 32, 32, 2], [68, 8, 8, 68, 68],[32, 2], [38, 38], [32, 19, 2],[53, 60, 44], [32, 17, 17, 2],[16, 16, 31, 31]);txt = getActiveGroup(gcbh);text(2, 100, txt,'verticalAlignment', 'top');
  Sum : Sum
  "Target flag " : If  NumInputs=2  IfExpression=(u1>u2)  ElseIfExpressions=(u1<0)
  To Workspace : ToWorkspace  VariableName=V_host  SaveFormat=Timeseries  SampleTime=-1
  To Workspace1 : ToWorkspace  VariableName=V_target  SaveFormat=Timeseries  SampleTime=-1
  To Workspace2 : ToWorkspace  VariableName=Target_x  SaveFormat=Timeseries  SampleTime=-1
  To Workspace3 : ToWorkspace  VariableName=Host_x  SaveFormat=Timeseries  SampleTime=-1
  To Workspace4 : ToWorkspace  VariableName=Range_rate  SaveFormat=Timeseries  SampleTime=-1
  To Workspace5 : ToWorkspace  VariableName=Range  SaveFormat=Timeseries  SampleTime=-1
  Range_Rate_mps : Outport
  R_target : Outport  Port=2
  R_host : Outport  Port=3
  Range_m : Outport  Port=4
  Target_flag : Outport  Port=5
  wires:
  Integrator1/1 -> R_host/1, [R_host]  "R_host"
  Integrator/1 -> [R_target], R_target/1  "R_target"
  Merge/1 -> Scope/1, Manual Switch/2
  "Target flag "/1 -> If Action Subsystem/Action
  "Target flag "/3 -> If Action Subsystem1/Action
  Range_threshold/1 -> "Target flag "/2
  [V_host_mps] -> Integrator1/1
  [R_host] -> Add/2
  V_host_mps/1 -> [V_host_mps], Sum/2  "V_host"
  [R_target] -> Add/1
  [V_target_mps] -> Integrator/1
  Sum/1 -> [Range_rate_mps], Range_Rate_mps/1  "Range_rate_mps"
  Add/1 -> [Range_m], Range_m/1  "Range_m"
  V_target_mps/1 -> [V_target_mps], Sum/1  "v_target"
  [Range_m] -> "Target flag "/1
  Manual Switch/1 -> Scope1/1, Target_flag/1
  Constant1/1 -> Integrator/2
  Constant2/1 -> Integrator1/2
  "Target flag "/2 -> If Action Subsystem2/Action
  If Action Subsystem/1(Output) -> Merge/1
  If Action Subsystem2/1(Output) -> Merge/2
  If Action Subsystem1/1(Output) -> Merge/3
  [V_host_mps] -> Scope2/1, To Workspace/1
  [V_target_mps] -> To Workspace1/1, Scope2/2
  [R_target] -> Scope3/1, To Workspace2/1
  [R_host] -> To Workspace3/1, Scope3/2
  [Range_rate_mps] -> Scope4/1, To Workspace4/1
  [Range_m] -> Scope4/2, To Workspace5/1
  Signal Builder/2(no target) -> Manual Switch1/2
  Signal Builder/1(target) -> Manual Switch1/1
  Manual Switch1/1 -> Manual Switch/1

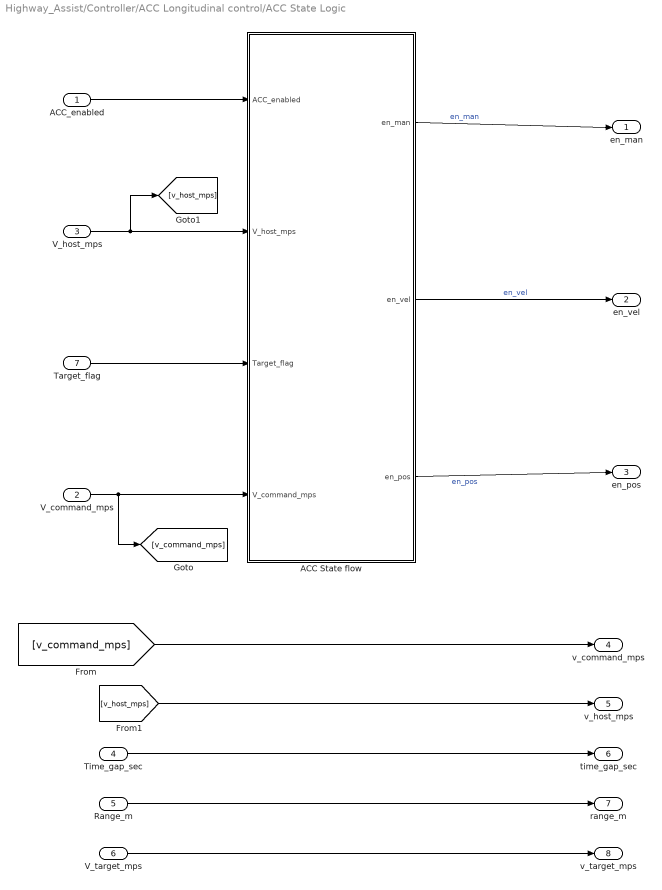
== system Highway_Assist/Controller/ACC Longitudinal control/ACC State Logic ==
  ACC_enabled : Inport
  V_command_mps : Inport  Port=2
  V_host_mps : Inport  Port=3
  Time_gap_sec : Inport  Port=4
  Range_m : Inport  Port=5
  V_target_mps : Inport  Port=6
  Target_flag : Inport  Port=7
  ACC State flow : Stateflow chart  TreatAsAtomicUnit=on
  en_man : Outport
  en_vel : Outport  Port=2
  en_pos : Outport  Port=3
  v_command_mps : Outport  Port=4
  v_host_mps : Outport  Port=5
  time_gap_sec : Outport  Port=6
  range_m : Outport  Port=7
  v_target_mps : Outport  Port=8
  wires:
  ACC State flow/2(en_vel) -> en_vel/1  "en_vel"
  ACC State flow/3(en_pos) -> en_pos/1  "en_pos"
  [v_command_mps] -> v_command_mps/1
  [v_host_mps] -> v_host_mps/1
  Time_gap_sec/1 -> time_gap_sec/1
  Range_m/1 -> range_m/1
  V_target_mps/1 -> v_target_mps/1
  ACC State flow/1(en_man) -> en_man/1  "en_man"
  ACC_enabled/1 -> ACC State flow/1(ACC_enabled)
  Target_flag/1 -> ACC State flow/3(Target_flag)
  V_host_mps/1 -> [v_host_mps], ACC State flow/2(V_host_mps)
  V_command_mps/1 -> ACC State flow/4(V_command_mps), [v_command_mps]

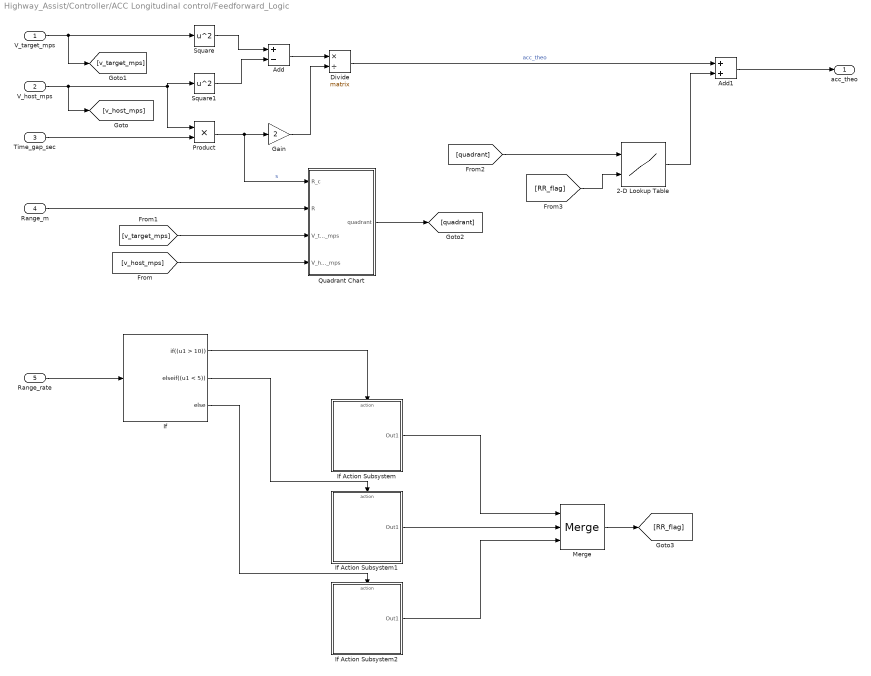
== system Highway_Assist/Controller/ACC Longitudinal control/Feedforward_Logic ==
  V_target_mps : Inport
  V_host_mps : Inport  Port=2
  Time_gap_sec : Inport  Port=3
  Range_m : Inport  Port=4
  Range_rate : Inport  Port=5
  2-D Lookup Table : Lookup_n-D  BreakpointsForDimension1=[1,2,3,4]  BreakpointsForDimension2=[1,2,3]  Table=reshape([50,1,60,60,40,1,70,70,20,1,80,80],4,3)  InternalRulePriority=Speed  RndMeth=Simplest  InputSameDT=on
      settings: InputPortMap=u0,u1
  Add : Sum  Inputs=+-
  Add1 : Sum
  Divide : Product  Inputs=*/  Multiplication=Matrix(*)
  Gain : Gain  Gain=2
  If : If  IfExpression=(u1 > 10)  ElseIfExpressions=(u1 < 5)
  If Action Subsystem : Subsystem  TreatAsAtomicUnit=on
  If Action Subsystem1 : Subsystem  TreatAsAtomicUnit=on
  If Action Subsystem2 : Subsystem  TreatAsAtomicUnit=on
  Merge : Merge  Inputs=3
  Product : Product
  Quadrant Chart : Stateflow chart  TreatAsAtomicUnit=on
  Square : Math  Operator=square  SaturateOnIntegerOverflow=on
  Square1 : Math  Operator=square  SaturateOnIntegerOverflow=on
  acc_theo : Outport
  wires:
  V_target_mps/1 -> [v_target_mps], Square/1
  V_host_mps/1 -> [v_host_mps], Square1/1, Product/1
  Square/1 -> Add/1
  Square1/1 -> Add/2
  Time_gap_sec/1 -> Product/2
  Product/1 -> Quadrant Chart/1(R_c), Gain/1  "s"
  Add/1 -> Divide/1
  Gain/1 -> Divide/2
  Divide/1 -> Add1/1  "acc_theo"
  Range_m/1 -> Quadrant Chart/2(R)
  [v_host_mps] -> Quadrant Chart/4(V_host_mps)
  [v_target_mps] -> Quadrant Chart/3(V_target_mps)
  Quadrant Chart/1(quadrant) -> [quadrant]
  [quadrant] -> 2-D Lookup Table/1
  If/1 -> If Action Subsystem/Action
  If/2 -> If Action Subsystem1/Action
  If/3 -> If Action Subsystem2/Action
  Range_rate/1 -> If/1
  If Action Subsystem1/1(Out1) -> Merge/2
  If Action Subsystem/1(Out1) -> Merge/1
  If Action Subsystem2/1(Out1) -> Merge/3
  Merge/1 -> [RR_flag]
  [RR_flag] -> 2-D Lookup Table/2
  2-D Lookup Table/1 -> Add1/2
  Add1/1 -> acc_theo/1

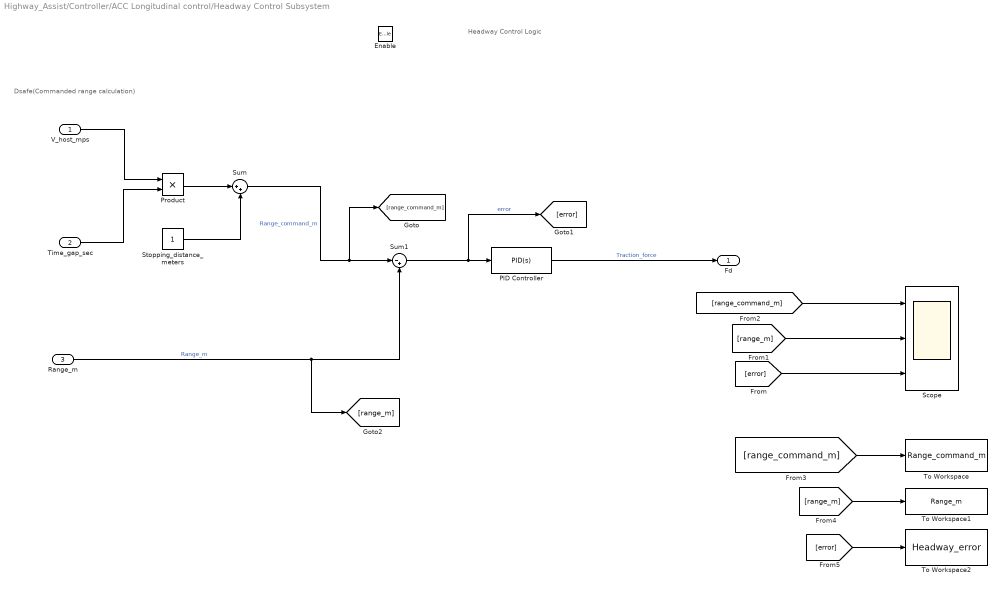
== system Highway_Assist/Controller/ACC Longitudinal control/Headway Control Subsystem ==
  note: Headway Control Logic
  note: Dsafe(Commanded range calculation)
  V_host_mps : Inport
  Time_gap_sec : Inport  Port=2
  Range_m : Inport  Port=3
  Enable : EnablePort
  PID Controller : pid_lib/PID Controller  Controller=PID  Form=Parallel  TimeDomain=Continuous-time  UseExternalTs=off  SampleTime=-1  IntegratorMethod=Forward Euler  FilterMethod=Forward Euler  ControllerParametersSource=internal  P=1.23373996546318  I=0.00611903694432425  D=34.7378082281947  UseFilter=on  N=75  TunerSelectOption=Transfer Function Based (PID Tuner App)  InitialConditionSource=internal  InitialConditionForIntegrator=0  InitialConditionForFilter=0  DifferentiatorICPrevScaledInput=0  ExternalReset=none  TrackingMode=off  Kt=1  LimitOutput=off  SatLimitsSource=internal  UpperSaturationLimit=inf  LowerSaturationLimit=-inf  LinearizeAsGain=on  AntiWindupMode=none  Kb=1  POutMin=[]  POutMax=[]  IOutMin=[]  IOutMax=[]  DOutMin=[]  DOutMax=[]  NOutMin=[]  NOutMax=[]  SumOutMin=[]  SumOutMax=[]  SaturationOutMin=[]  SaturationOutMax=[]  PParamMin=[]  PParamMax=[]  IParamMin=[]  IParamMax=[]  DParamMin=[]  DParamMax=[]  NParamMin=[]  NParamMax=[]  KbParamMin=[]  KbParamMax=[]  KtParamMin=[]  KtParamMax=[]  KbOutMin=[]  KbOutMax=[]  KtOutMin=[]  KtOutMax=[]  IntegratorOutMin=[]  IntegratorOutMax=[]  FilterOutMin=[]  FilterOutMax=[]  SumI1OutMin=[]  SumI1OutMax=[]  SumI2OutMin=[]  SumI2OutMax=[]  SumI3OutMin=[]  SumI3OutMax=[]  SumI4OutMin=[]  SumI4OutMax=[]  SumDOutMin=[]  SumDOutMax=[]  DifferentiatorOutMin=[]  DifferentiatorOutMax=[]  FilterDiffOutCoefMin=[]  FilterDiffOutCoefMax=[]  ReciprocalOutMin=[]  ReciprocalOutMax=[]  SumDenOutMin=[]  SumDenOutMax=[]  SumNumOutMin=[]  SumNumOutMax=[]  DivideOutMin=[]  DivideOutMax=[]  UdiffTsProdOutMin=[]  UdiffTsProdOutMax=[]  NTsProdOutMin=[]  NTsProdOutMax=[]  UintegralTsProdOutMin=[]  UintegralTsProdOutMax=[]  UngainTsProdOutMin=[]  UngainTsProdOutMax=[]  IntegratorContinuousStateAttributes=''  IntegratorStateMustResolveToSignalObject=off  IntegratorRTWStateStorageClass=Auto  FilterContinuousStateAttributes=''  FilterStateMustResolveToSignalObject=off  FilterRTWStateStorageClass=Auto  ParallelPVariant=InternalParameters  IdealPVariant=Disabled  IVariant=InternalParameters  DVariant=InternalParameters  IntegratorVariant=Continuous  SatVariant=Disabled  AWVariant=Passthrough  PCopyVariant=Disabled  TRVariant=Disabled  FdbkBlocksVariant=Forward  IdealPFdbkVariant=Disabled  SatFdbkVariant=Disabled  DerivativeFilterVariant=ContFilter  NVariant=InternalParameters  NCopyVariant=Disabled  FilterICVariant=InternalICsFilter  IntegratorICVariant=InternalICs  ExternalResetVariant=Disabled  TRSumVariant=Passthrough  SumFdbkVariant=Disabled  SumVariant=Sum_PID  TsampFilterVariant=InternalTs  TsampNgainVariant=Passthrough  TsampIntegralVariant=Passthrough  ExternalSaturationOutDataTypeStr=Inherit: Same as second input
  Product : Product
  Scope : Scope  NumInputPorts=3
  Stopping_distance_meters : Constant
  Sum : Sum  Inputs=|++
  Sum1 : Sum  Inputs=|-+
  To Workspace : ToWorkspace  VariableName=Range_command_m  SampleTime=-1
  To Workspace1 : ToWorkspace  VariableName=Range_m  SampleTime=-1
  To Workspace2 : ToWorkspace  VariableName=Headway_error  SaveFormat=Timeseries  SampleTime=-1
  Fd : Outport
  wires:
  [range_m] -> To Workspace1/1
  [error] -> Scope/3
  [error] -> To Workspace2/1
  [range_command_m] -> Scope/1
  [range_m] -> Scope/2
  [range_command_m] -> To Workspace/1
  PID Controller/1 -> Fd/1  "Traction_force"
  Sum/1 -> [range_command_m], Sum1/1  "Range_command_m"
  Stopping_distance_meters/1 -> Sum/2
  V_host_mps/1 -> Product/1
  Sum1/1 -> [error], PID Controller/1  "error"
  Time_gap_sec/1 -> Product/2
  Range_m/1 -> [range_m], Sum1/2  "Range_m"
  Product/1 -> Sum/1

== system Highway_Assist/Controller/ACC Longitudinal control/Manual Mode Subsystem ==
  Fd_throttle : Inport
  Enable : EnablePort
  Fd : Outport
  wires:
  Fd_throttle/1 -> Fd/1

== system Highway_Assist/Controller/ACC Longitudinal control/Velocity Control Subsystem ==
  V_command_mps : Inport
  V_host_mps : Inport  Port=2
  Enable : EnablePort
  PID Controller : pid_lib/PID Controller  Controller=PID  Form=Parallel  TimeDomain=Continuous-time  UseExternalTs=off  SampleTime=-1  IntegratorMethod=Forward Euler  FilterMethod=Forward Euler  ControllerParametersSource=internal  P=174.6119  I=10.1187  D=247.7833  UseFilter=on  N=100  TunerSelectOption=Transfer Function Based (PID Tuner App)  InitialConditionSource=internal  InitialConditionForIntegrator=0  InitialConditionForFilter=0  DifferentiatorICPrevScaledInput=0  ExternalReset=none  TrackingMode=off  Kt=1  LimitOutput=off  SatLimitsSource=internal  UpperSaturationLimit=inf  LowerSaturationLimit=-inf  LinearizeAsGain=on  AntiWindupMode=none  Kb=1  POutMin=[]  POutMax=[]  IOutMin=[]  IOutMax=[]  DOutMin=[]  DOutMax=[]  NOutMin=[]  NOutMax=[]  SumOutMin=[]  SumOutMax=[]  SaturationOutMin=[]  SaturationOutMax=[]  PParamMin=[]  PParamMax=[]  IParamMin=[]  IParamMax=[]  DParamMin=[]  DParamMax=[]  NParamMin=[]  NParamMax=[]  KbParamMin=[]  KbParamMax=[]  KtParamMin=[]  KtParamMax=[]  KbOutMin=[]  KbOutMax=[]  KtOutMin=[]  KtOutMax=[]  IntegratorOutMin=[]  IntegratorOutMax=[]  FilterOutMin=[]  FilterOutMax=[]  SumI1OutMin=[]  SumI1OutMax=[]  SumI2OutMin=[]  SumI2OutMax=[]  SumI3OutMin=[]  SumI3OutMax=[]  SumI4OutMin=[]  SumI4OutMax=[]  SumDOutMin=[]  SumDOutMax=[]  DifferentiatorOutMin=[]  DifferentiatorOutMax=[]  FilterDiffOutCoefMin=[]  FilterDiffOutCoefMax=[]  ReciprocalOutMin=[]  ReciprocalOutMax=[]  SumDenOutMin=[]  SumDenOutMax=[]  SumNumOutMin=[]  SumNumOutMax=[]  DivideOutMin=[]  DivideOutMax=[]  UdiffTsProdOutMin=[]  UdiffTsProdOutMax=[]  NTsProdOutMin=[]  NTsProdOutMax=[]  UintegralTsProdOutMin=[]  UintegralTsProdOutMax=[]  UngainTsProdOutMin=[]  UngainTsProdOutMax=[]  IntegratorContinuousStateAttributes=''  IntegratorStateMustResolveToSignalObject=off  IntegratorRTWStateStorageClass=Auto  FilterContinuousStateAttributes=''  FilterStateMustResolveToSignalObject=off  FilterRTWStateStorageClass=Auto  ParallelPVariant=InternalParameters  IdealPVariant=Disabled  IVariant=InternalParameters  DVariant=InternalParameters  IntegratorVariant=Continuous  SatVariant=Disabled  AWVariant=Passthrough  PCopyVariant=Disabled  TRVariant=Disabled  FdbkBlocksVariant=Forward  IdealPFdbkVariant=Disabled  SatFdbkVariant=Disabled  DerivativeFilterVariant=ContFilter  NVariant=InternalParameters  NCopyVariant=Disabled  FilterICVariant=InternalICsFilter  IntegratorICVariant=InternalICs  ExternalResetVariant=Disabled  TRSumVariant=Passthrough  SumFdbkVariant=Disabled  SumVariant=Sum_PID  TsampFilterVariant=InternalTs  TsampNgainVariant=Passthrough  TsampIntegralVariant=Passthrough  ExternalSaturationOutDataTypeStr=Inherit: Same as second input
  Scope : Scope  NumInputPorts=2
  Sum : Sum  Inputs=|+-
  Fd : Outport
  wires:
  V_host_mps/1 -> Scope/2, Sum/2
  V_command_mps/1 -> Scope/1, Sum/1
  Sum/1 -> PID Controller/1
  PID Controller/1 -> Fd/1

== system Highway_Assist/Controller/MPC Lateral control/MPC ==
  note: LATERAL CONTROL WITH MPC
  seq_curvature : Inport
  V_host_mps : Inport  Port=2
  lateral_deviation : Inport  Port=3
  Relative_yaw_angle : Inport  Port=4
  Enable : EnablePort
  Lane Keeping Assist System : mpcadaslib/Lane Keeping Assist System  ModelType=Use vehicle parameters  VehicleMass=1140  VehicleYawInertia=1436.24  LengthToFront=1.165  LengthToRear=1.165  FrontTireStiffness=155494.663  RearTireStiffness=1554494.663  EgoModelMatrixA=[-4.4021 ,-12.4603;1.3913,-5.1868]  EgoModelMatrixB=[24.1270;15.8609]  EgoModelMatrixC=[1,0;0,1]  InitialLongVel=V_init  TransportLag=0  MinSteering=-0.5  umin_ext=off  MaxSteering=0.5  umax_ext=off  Ts=0.1  PredictionHorizon=10  ControllerBehavior=0.23999999999999999  suboptimal=off  maxiter=10  datatypeopt=double  optmode=off  trackmode=off
      settings: SourceProductBaseCode=MP
  Scope : Scope
  Scope1 : Scope  NumInputPorts=3
  To Workspace : ToWorkspace  VariableName=cross_track  SampleTime=-1
  To Workspace1 : ToWorkspace  VariableName=Theta_e  SampleTime=-1
  steering angle (rad) : Outport
  wires:
  seq_curvature/1 -> Lane Keeping Assist System/1
  Lane Keeping Assist System/1 -> steering angle (rad)/1, Scope/1
  V_host_mps/1 -> Scope1/1, Lane Keeping Assist System/2
  lateral_deviation/1 -> Scope1/2, Lane Keeping Assist System/3, To Workspace/1
  Relative_yaw_angle/1 -> To Workspace1/1, Scope1/3, Lane Keeping Assist System/4

== system Highway_Assist/Controller/MPC Lateral control/manual ==
  Enable : EnablePort
  Constant : Constant  Value=0
  delta : Outport
  wires:
  Constant/1 -> delta/1

== system Highway_Assist/Sensor inputs/Lateral control sensor inputs/Subsystem ==
  MATLAB Function : MATLAB Function  TreatAsAtomicUnit=on
  Memory1 : Memory  InheritSampleTime=on  LinearizeAsDelay=on
  sequence : Outport  VectorParamsAs1DForOutWhenUnconnected=off
  current : Outport  Port=2  VectorParamsAs1DForOutWhenUnconnected=off
  wires:
  MATLAB Function/2(first) -> current/1
  MATLAB Function/3(next_t) -> Memory1/1
  MATLAB Function/1(seq) -> sequence/1
  Memory1/1 -> MATLAB Function/1(t)

== system Highway_Assist/Sensor inputs/Lateral control sensor inputs/sensor dynamics ==
  note: The lateral deviation is the cross track error
  Current_curvature : Inport
  Longitudinal velocity : Inport  Port=2
  Lateral velocity : Inport  Port=3
  Yaw rate : Inport  Port=4
  Integrator : Integrator
  Integrator1 : Integrator
  Mux : Mux  Inputs=3
  Product : Product
  Sum : Sum  Inputs=+-
  Lateral deviation : Outport
  Relative yaw angle : Outport  Port=2
  wires:
  Longitudinal velocity/1 -> Product/1, Mux/3
  Current_curvature/1 -> Product/2
  Mux/1 -> Integrator1/1  "e1_dot"
  Integrator1/1 -> Lateral deviation/1  "e1"
  Yaw rate/1 -> Sum/1
  Product/1 -> Sum/2
  Sum/1 -> Integrator/1  "e2dot"
  Integrator/1 -> Mux/2, Relative yaw angle/1  "e2"
  Lateral velocity/1 -> Mux/1

== system Highway_Assist/Sensor inputs/Radar sensor output/If Action Subsystem ==
  Action Port : ActionPort  ActionPortLabel=if((u1>u2))
  Constant : Constant  Value=0
  Output : Outport
  wires:
  Constant/1 -> Output/1

== system Highway_Assist/Sensor inputs/Radar sensor output/If Action Subsystem1 ==
  Action Port : ActionPort  ActionPortLabel=else
  Constant : Constant
  Output : Outport
  wires:
  Constant/1 -> Output/1

== system Highway_Assist/Sensor inputs/Radar sensor output/If Action Subsystem2 ==
  Action Port : ActionPort  ActionPortLabel=elseif((u1<0))
  Constant : Constant  Value=0
  Output : Outport
  wires:
  Constant/1 -> Output/1
